simulink model "PV_SingleDiode_Model_v0_1"  (R2025b)
settings: Solver=ode23t  StartTime=0.0  StopTime=PVSDM.SweepTime  MaxStep=0.01  RelTol=1e-3
undefined symbols (not defined in the file or in its folder): PVSDM
libraries: simulink x1
settings Model: Creator=jamielangeveldt  LastModifiedBy=jamielangeveldt

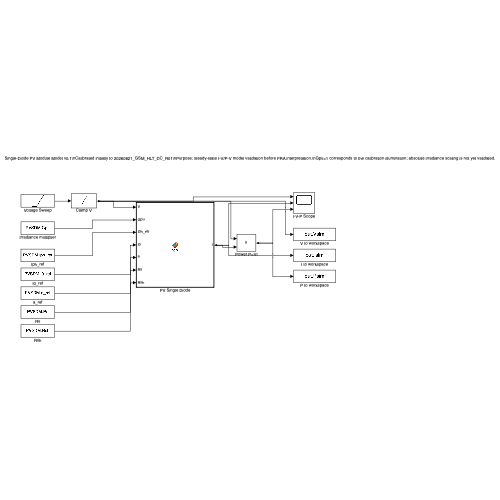
[thumbnail: Simulink's stored preview of the top-level diagram]
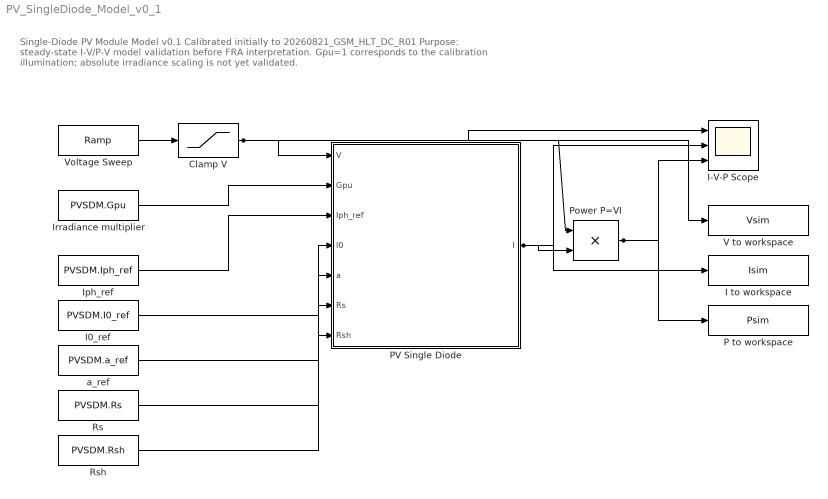
== system PV_SingleDiode_Model_v0_1 ==
  note: Single-Diode PV Module Model v0.1\nCalibrated initially to 20260821_GSM_HLT_DC_R01\nPurpose: steady-state I-V/P-V model validation before FRA interpretation.\nGpu=1 corresponds to the calibration illumination; absolute irradiance scaling is not yet validated.
  Clamp V : Saturate  UpperLimit=PVSDM.Vmax  LowerLimit=0
  I to workspace : ToWorkspace  VariableName=Isim  SaveFormat=Structure With Time  SampleTime=-1
  I-V-P Scope : Scope  NumInputPorts=3
  I0_ref : Constant  Value=PVSDM.I0_ref
  Iph_ref : Constant  Value=PVSDM.Iph_ref
  Irradiance multiplier : Constant  Value=PVSDM.Gpu
  P to workspace : ToWorkspace  VariableName=Psim  SaveFormat=Structure With Time  SampleTime=-1
  PV Single Diode : MATLAB Function  TreatAsAtomicUnit=on
  Power P=VI : Product
  Rs : Constant  Value=PVSDM.Rs
  Rsh : Constant  Value=PVSDM.Rsh
  V to workspace : ToWorkspace  VariableName=Vsim  SaveFormat=Structure With Time  SampleTime=-1
  Voltage Sweep : simulink/Sources/Ramp  slope=PVSDM.Vmax/PVSDM.SweepTime  start=0  InitialOutput=0
  a_ref : Constant  Value=PVSDM.a_ref
  wires:
  Voltage Sweep/1 -> Clamp V/1
  Clamp V/1 -> PV Single Diode/1(V), Power P=VI/1, I-V-P Scope/1, V to workspace/1
  Irradiance multiplier/1 -> PV Single Diode/2(Gpu)
  Iph_ref/1 -> PV Single Diode/3(Iph_ref)
  I0_ref/1 -> PV Single Diode/4(I0)
  a_ref/1 -> PV Single Diode/5(a)
  Rs/1 -> PV Single Diode/6(Rs)
  Rsh/1 -> PV Single Diode/7(Rsh)
  PV Single Diode/1(I) -> Power P=VI/2, I-V-P Scope/2, I to workspace/1
  Power P=VI/1 -> I-V-P Scope/3, P to workspace/1

== matlab function PV_SingleDiode_Model_v0_1/PV Single Diode ==
  data: V input; I output; Gpu input; Iph_ref input; I0 input; a input; Rs input; Rsh input
function I = fcn(V,Gpu,Iph_ref,I0,a,Rs,Rsh)
%#codegen
% Implicit single-diode module equation solved by Newton iteration.
% Gpu is relative irradiance; 1.0 = calibration illumination.
Iph = max(0, Iph_ref*Gpu);
I = Iph;
for k = 1:20
    arg = (V + I*Rs)/max(a,1e-9);
    arg = min(max(arg,-50),50);
    ea = exp(arg);
    F = I - Iph + I0*(ea - 1) + (V + I*Rs)/max(Rsh,1e-9);
    dF = 1 + I0*ea*(Rs/max(a,1e-9)) + Rs/max(Rsh,1e-9);
    step = F/max(dF,1e-12);
    step = min(max(step,-0.5),0.5);
    I = I - step;
end
end
